simulink subsystem "Supervisor"  (R2024a)
settings: Solver=VariableStepAuto  StartTime=0.0  StopTime=10.0  RelTol=1e-3
settings Model: Creator=User  LastModifiedBy=User

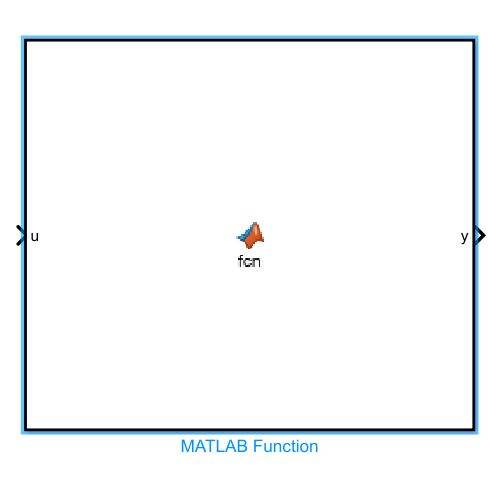
[thumbnail: Simulink's stored preview of the top-level diagram]
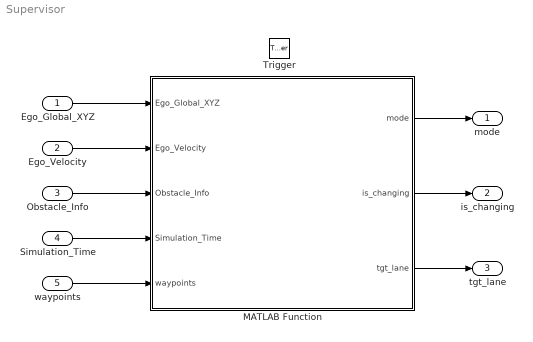
== system Supervisor ==
  Ego_Global_XYZ : Inport
  Ego_Velocity : Inport  Port=2
  Obstacle_Info : Inport  Port=3
  Simulation_Time : Inport  Port=4
  waypoints : Inport  Port=5
  Trigger : TriggerPort  TriggerType=function-call  VariantControl=(inherit)  PortDimensions=1
  MATLAB Function : MATLAB Function  TreatAsAtomicUnit=on
  mode : Outport
  is_changing : Outport  Port=2
  tgt_lane : Outport  Port=3
  wires:
  Ego_Global_XYZ/1 -> MATLAB Function/1(Ego_Global_XYZ)
  Ego_Velocity/1 -> MATLAB Function/2(Ego_Velocity)
  Obstacle_Info/1 -> MATLAB Function/3(Obstacle_Info)
  Simulation_Time/1 -> MATLAB Function/4(Simulation_Time)
  waypoints/1 -> MATLAB Function/5(waypoints)
  MATLAB Function/1(mode) -> mode/1
  MATLAB Function/2(is_changing) -> is_changing/1
  MATLAB Function/3(tgt_lane) -> tgt_lane/1

== matlab function Supervisor/MATLAB Function ==
  data: mode output; is_changing output; tgt_lane output; Ego_Global_XYZ input; Ego_Velocity input; Obstacle_Info input; Simulation_Time input; waypoints input
function [mode, is_changing, tgt_lane]= Superviosr(Ego_Global_XYZ, Ego_Velocity, Obstacle_Info, Simulation_Time, waypoints)
